simulink model "zsi_mppt_grid_pv"  (R2024b)
settings: Solver=FixedStepDiscrete  StartTime=0.0  StopTime=5  FixedStep=1e-6  RelTol=1e-3
libraries: spsSeriesRLCBranchLib x5, spsDiodeLib x4, spsVoltageMeasurementLib x4, spsPVArrayLib x3, dspstat3 x2, spsCurrentMeasurementLib x1, simulink x1, spsThreePhaseSeriesRLCBranchLib x1, spsThreePhaseVIMeasurementLib x1, spsThreePhaseSourceLib x1, spsUniversalBridgeLib x1, sps_lib x1
settings Model: Creator=Dhananjay Dhumal  LastModifiedBy=Dhananjay Dhumal
settings DebuggingCC: SignalInfNanChecking=error

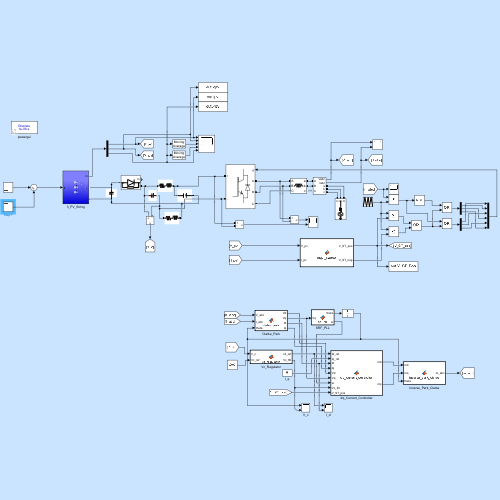
[thumbnail: Simulink's stored preview of the top-level diagram]
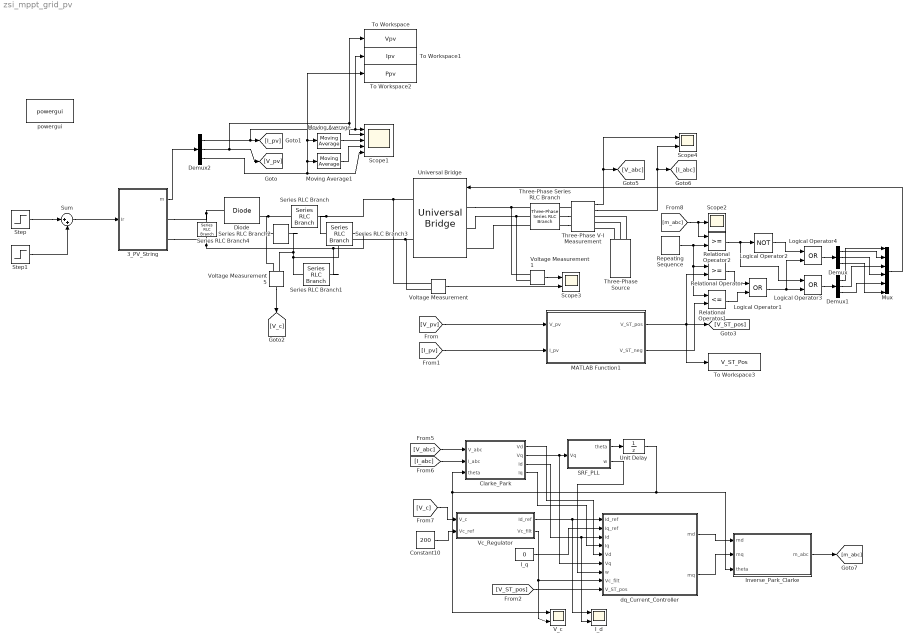
== system zsi_mppt_grid_pv ==
  3_PV_String : Subsystem
  Clarke_Park : MATLAB Function  TreatAsAtomicUnit=on
  Constant10 : Constant  Value=200
  Demux : Demux  Outputs=3
  Demux1 : Demux  Outputs=3
  Demux2 : Demux  Outputs=3
  Diode : spsDiodeLib/Diode  Ron=0.001  Lon=0  Vf=0.8  IC=0  UseSnubber=0  Rs=500  Cs=250e-9  Measurements=on
  I_d : Scope  NumInputPorts=2
  I_q : Constant  Value=0
  Inverse_Park_Clarke : MATLAB Function  TreatAsAtomicUnit=on
  Logical Operator1 : Logic  Operator=OR  AllPortsSameDT=off  OutDataTypeStr=boolean
  Logical Operator2 : Logic  Operator=NOT  AllPortsSameDT=off  OutDataTypeStr=boolean
  Logical Operator3 : Logic  Operator=OR  AllPortsSameDT=off  OutDataTypeStr=boolean
  Logical Operator4 : Logic  Operator=OR  AllPortsSameDT=off  OutDataTypeStr=boolean
  MATLAB Function1 : MATLAB Function  TreatAsAtomicUnit=on
  Moving Average : dspstat3/Moving Average  Method=Sliding window  ForgettingFactorPort=off  SpecifyWindowLength=on  WindowLength=500  OverlapLength=499  AllowArbitraryInputLength=off  ForgettingFactor=0.9  SimulateUsing=Interpreted execution
  Moving Average1 : dspstat3/Moving Average  Method=Sliding window  ForgettingFactorPort=off  SpecifyWindowLength=on  WindowLength=10000  OverlapLength=9999  AllowArbitraryInputLength=off  ForgettingFactor=0.9  SimulateUsing=Interpreted execution
  Mux : Mux  Inputs=6
  Relational Operator : RelationalOperator  OutDataTypeStr=boolean  RndMeth=Simplest  InputSameDT=off
  Relational Operator1 : RelationalOperator  Operator=<=  OutDataTypeStr=boolean  RndMeth=Simplest  InputSameDT=off
  Relational Operator2 : RelationalOperator  OutDataTypeStr=boolean  RndMeth=Simplest  InputSameDT=off
  Repeating Sequence : simulink/Sources/Repeating Sequence  rep_seq_t=[0 0.5e-4 1e-4]  rep_seq_y=[-1 1 -1]
  SRF_PLL : MATLAB Function  TreatAsAtomicUnit=on
  Scope1 : Scope  NumInputPorts=5
  Scope2 : Scope
  Scope3 : Scope  NumInputPorts=2
  Scope4 : Scope  NumInputPorts=2
  Series RLC Branch : spsSeriesRLCBranchLib/Series RLC Branch  LConnTagsString=__new0  RConnTagsString=__new0  BranchType=RL  Resistance=0.2  Inductance=1e-3  SetiL0=off  InitialCurrent=0  Capacitance=1e-6  Setx0=off  InitialVoltage=0  Measurements=None
  Series RLC Branch1 : spsSeriesRLCBranchLib/Series RLC Branch  LConnTagsString=__new0  RConnTagsString=__new0  BranchType=RL  Resistance=0.2  Inductance=1e-3  SetiL0=off  InitialCurrent=0  Capacitance=1e-6  Setx0=off  InitialVoltage=0  Measurements=None
  Series RLC Branch2 : spsSeriesRLCBranchLib/Series RLC Branch  LConnTagsString=__new0  RConnTagsString=__new0  BranchType=C  Resistance=1  Inductance=1e-3  SetiL0=off  InitialCurrent=0  Capacitance=1000e-6  Setx0=on  InitialVoltage=200  Measurements=None
  Series RLC Branch3 : spsSeriesRLCBranchLib/Series RLC Branch  LConnTagsString=__new0  RConnTagsString=__new0  BranchType=C  Resistance=1  Inductance=1000e-3  SetiL0=off  InitialCurrent=0  Capacitance=1000e-6  Setx0=on  InitialVoltage=200  Measurements=None
  Series RLC Branch4 : spsSeriesRLCBranchLib/Series RLC Branch  LConnTagsString=__new0  RConnTagsString=__new0  BranchType=C  Resistance=1  Inductance=1e-3  SetiL0=off  InitialCurrent=0  Capacitance=150e-6  Setx0=on  InitialVoltage=192  Measurements=None
  Step : Step  Time=1.5  Before=[1000, 1000, 1000]  After=[1000, 700, 350]  SampleTime=0
  Step1 : Step  Time=3.5  Before=[0, 0, 0]  After=[-800, -200, 700]  SampleTime=0
  Sum : Sum  Inputs=|++
  Three-Phase Series RLC Branch : spsThreePhaseSeriesRLCBranchLib/Three-Phase Series RLC Branch  LConnTagsString=A|B|C  RConnTagsString=A|B|C  BranchType=L  Resistance=1  Inductance=5e-3  Capacitance=1e-6  Measurements=None
  Three-Phase V-I Measurement : spsThreePhaseVIMeasurementLib/Three-Phase V-I Measurement  VoltageMeasurement=phase-to-ground  SetLabelV=off  LabelV=Vabc  Vpu=off  VpuLL=off  CurrentMeasurement=yes  SetLabelI=off  LabelI=Iabc  Ipu=off  Pbase=100e6  Vbase=500e3  OutputType=Complex  PhasorSimulation=off  PSBequivalent=0
  Three-Phase Source : spsThreePhaseSourceLib/Three-Phase Source  InternalConnection=Yg  VoltagePhases=off  Voltage=100  PhaseAngle=0  Voltage_phases=[25e3 25e3 25e3]/sqrt(3)  PhaseAngles_phases=[0 -120 +120]  Frequency=50  NonIdealSource=on  SpecifyImpedance=off  Resistance=0.001  Inductance=0  ShortCircuitLevel=100e6  BaseVoltage=100  XRratio=7  BusType=swing  Pref=10e3  Qref=0  Prefabc=[10e3, 10e3, 10e3]  Qrefabc=[0, 0, 0]  Qmin=-inf  Qmax=inf
  To Workspace : ToWorkspace  VariableName=Vpv  SaveFormat=Timeseries  SampleTime=-1
  To Workspace1 : ToWorkspace  VariableName=Ipv  SaveFormat=Timeseries  SampleTime=-1
  To Workspace2 : ToWorkspace  VariableName=Ppv  SaveFormat=Timeseries  SampleTime=-1
  To Workspace3 : ToWorkspace  VariableName=V_ST_Pos  SaveFormat=Timeseries  SampleTime=-1
  Unit Delay : UnitDelay  SampleTime=1e-6  HasFrameUpgradeWarning=on
  Universal Bridge : spsUniversalBridgeLib/Universal Bridge  Arms=3  SnubberResistance=1e5  SnubberCapacitance=inf  Device=IGBT / Diodes  Ron=1e-3  Lon=0  ForwardVoltages="[  0  0  ]"  ForwardVoltage=0  GTOparameters=[ 10e-6 , 20e-6 ]  IGBTparameters=[ 1e-6 , 2e-6 ]  Measurements=All voltages and currents  Measurements_2=None  converterType=Rectifier
  V_c : Scope  NumInputPorts=2
  Vc_Regulator : MATLAB Function  TreatAsAtomicUnit=on
  Voltage Measurement : spsVoltageMeasurementLib/Voltage Measurement  PhasorSimulation=off  OutputType=Complex  PSBequivalent=0
  Voltage Measurement1 : spsVoltageMeasurementLib/Voltage Measurement  PhasorSimulation=off  OutputType=Complex  PSBequivalent=0
  Voltage Measurement5 : spsVoltageMeasurementLib/Voltage Measurement  PhasorSimulation=off  OutputType=Complex  PSBequivalent=0
  dq_Current_Controller : MATLAB Function  TreatAsAtomicUnit=on
  powergui : sps_lib/powergui  Priority=1  SimulationMode=Discrete  SampleTime=1e-6  frequency=60  Iterations=50  frequencyindice=0  Pbase=100e6  ErrMax=1e-4  UnitsV=kV  UnitsW=MW  buscounter=0  FunctionMessages=off  echomessages=off  EnableUseOfTLC=off  CurrentSourceSwitches=off  DisableSnubberDevices=off  DisableRonSwitches=off  DisableVfSwitches=off  DisplayEquations=off  AutomaticDiscreteSolvers=off  SolverType=Tustin/Backward Euler (TBE)  Interpol=off  ExternalGateDelay=off  methode=off  Ts=100  x0status=blocks  SPID=on  SwTol=0  HookPort=off  NonlinearTolerance=1e-4  nMaxIteration=100  ContinueOnMaxIteration=off  RestoreLinks=warning  ResistiveCurrentMeasurement=off  Frange=[0:2:500]  Ylog=off  Xlog=on  ShowGrid=off  save=off  variable=ZData  structure=0  ZoomFFT=off  StartTime=0.0  cycles=1  DisplayStyle=1  fundamental=60  FreqAxis=off  MaxFrequency=1000  frequencyindicesteady=1  RmsSteady=1  display=off
  wires:
  Voltage Measurement/1 -> Scope3/2
  Repeating Sequence/1 -> Relational Operator2/2, Relational Operator/1, Relational Operator1/1
  Relational Operator/1 -> Logical Operator1/1
  Relational Operator1/1 -> Logical Operator1/2
  Logical Operator1/1 -> Logical Operator4/2, Logical Operator3/2
  Logical Operator4/1 -> Demux/1
  Logical Operator3/1 -> Demux1/1
  Voltage Measurement1/1 -> Scope3/1
  MATLAB Function1/1(V_ST_pos) -> To Workspace3/1, Relational Operator/2, [V_ST_pos]
  MATLAB Function1/2(V_ST_neg) -> Relational Operator1/2
  Voltage Measurement5/1 -> [V_c]
  Three-Phase V-I Measurement/1 -> Scope4/1, [V_abc]
  Three-Phase V-I Measurement/2 -> Scope4/2, [I_abc]
  [V_abc] -> Clarke_Park/1(V_abc)
  [I_abc] -> Clarke_Park/2(I_abc)
  Clarke_Park/2(Vq) -> dq_Current_Controller/6(Vq), SRF_PLL/1(Vq)
  SRF_PLL/1(theta) -> Unit Delay/1
  Unit Delay/1 -> V_c/1, Clarke_Park/3(theta), Inverse_Park_Clarke/3(theta)
  [V_c] -> Vc_Regulator/1(V_c)
  Constant10/1 -> Vc_Regulator/2(Vc_ref)
  Vc_Regulator/1(Id_ref) -> I_d/1, dq_Current_Controller/1(Id_ref)
  I_q/1 -> dq_Current_Controller/2(Iq_ref)
  Clarke_Park/3(Id) -> I_d/2, dq_Current_Controller/3(Id)
  Clarke_Park/4(Iq) -> dq_Current_Controller/4(Iq)
  Clarke_Park/1(Vd) -> dq_Current_Controller/5(Vd)
  SRF_PLL/2(w) -> dq_Current_Controller/7(w)
  Vc_Regulator/2(Vc_filt) -> V_c/2, dq_Current_Controller/8(Vc_filt)
  dq_Current_Controller/1(md) -> Inverse_Park_Clarke/1(md)
  dq_Current_Controller/2(mq) -> Inverse_Park_Clarke/2(mq)
  Inverse_Park_Clarke/1(m_abc) -> [m_abc]
  [m_abc] -> Scope2/1, Relational Operator2/1
  [V_ST_pos] -> dq_Current_Controller/9(V_ST_pos)
  [V_pv] -> MATLAB Function1/1(V_pv)
  [I_pv] -> MATLAB Function1/2(I_pv)
  Mux/1 -> Universal Bridge/1
  Relational Operator2/1 -> Logical Operator3/1, Logical Operator2/1
  Demux/1 -> Mux/2
  Demux/2 -> Mux/4
  Demux/3 -> Mux/6
  Demux1/1 -> Mux/1
  Demux1/2 -> Mux/3
  Demux1/3 -> Mux/5
  Logical Operator2/1 -> Logical Operator4/1
  Step/1 -> Sum/1
  3_PV_String/1(m) -> Demux2/1
  Demux2/1 -> To Workspace1/1, Scope1/1, [I_pv]
  Demux2/2 -> To Workspace/1, Scope1/2, [V_pv]
  Demux2/3 -> To Workspace2/1, Moving Average/1, Moving Average1/1, Scope1/5
  Moving Average/1 -> Scope1/3
  Moving Average1/1 -> Scope1/4
  Sum/1 -> 3_PV_String/1(Ir)
  Step1/1 -> Sum/2
  connections:
  Series RLC Branch/LConn1 -- Series RLC Branch2/LConn1 -- Voltage Measurement5/LConn1 -- Diode/RConn1
  Series RLC Branch3/RConn1 -- Series RLC Branch1/RConn1 -- 3_PV_String/RConn2 -- Series RLC Branch4/RConn1
  Series RLC Branch2/RConn1 -- Series RLC Branch1/LConn1 -- Voltage Measurement/LConn2 -- Universal Bridge/RConn2 -- Voltage Measurement5/LConn2
  Series RLC Branch/RConn1 -- Series RLC Branch3/LConn1 -- Universal Bridge/RConn1 -- Voltage Measurement/LConn1
  Universal Bridge/LConn1 -- Three-Phase Series RLC Branch/LConn1 -- Voltage Measurement1/LConn1
  Voltage Measurement1/LConn2 -- Three-Phase Series RLC Branch/LConn2 -- Universal Bridge/LConn2
  Three-Phase Series RLC Branch/LConn3 -- Universal Bridge/LConn3
  Three-Phase V-I Measurement/LConn1 -- Three-Phase Series RLC Branch/RConn1
  Three-Phase Series RLC Branch/RConn3 -- Three-Phase V-I Measurement/LConn3
  Three-Phase Series RLC Branch/RConn2 -- Three-Phase V-I Measurement/LConn2
  Three-Phase Source/RConn2 -- Three-Phase V-I Measurement/RConn2
  Three-Phase Source/RConn1 -- Three-Phase V-I Measurement/RConn1
  Three-Phase Source/RConn3 -- Three-Phase V-I Measurement/RConn3
  3_PV_String/RConn1 -- Diode/LConn1 -- Series RLC Branch4/LConn1

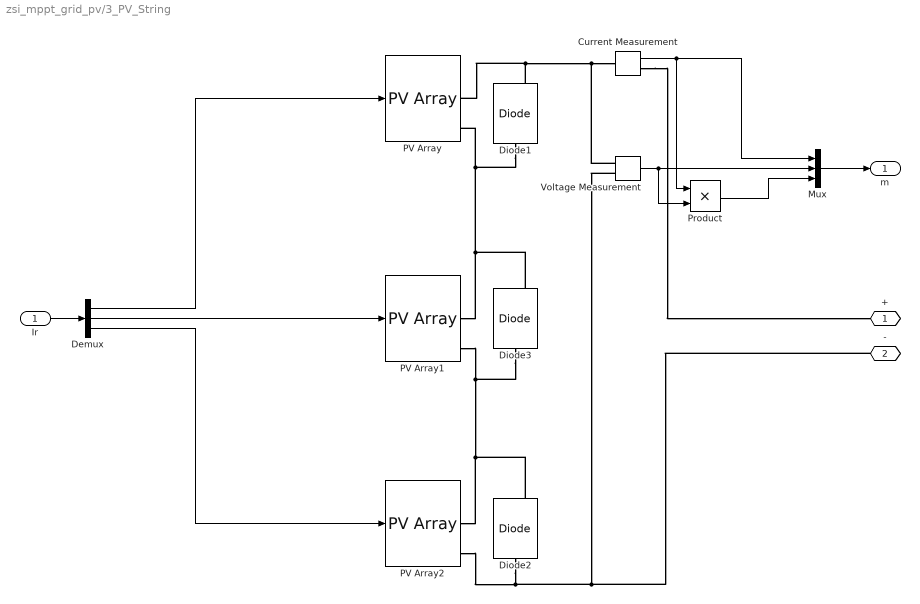
== system zsi_mppt_grid_pv/3_PV_String ==
  Ir : Inport  PortDimensions=3
  Current Measurement : spsCurrentMeasurementLib/Current Measurement  PhasorSimulation=off  OutputType=Complex  PSBequivalent=0
  Demux : Demux  Outputs=3
  Diode1 : spsDiodeLib/Diode  Ron=1e-5  Lon=0  Vf=0  IC=0  UseSnubber=0  Rs=1e5  Cs=inf  Measurements=on
  Diode2 : spsDiodeLib/Diode  Ron=1e-5  Lon=0  Vf=0  IC=0  UseSnubber=0  Rs=1e5  Cs=inf  Measurements=on
  Diode3 : spsDiodeLib/Diode  Ron=1e-5  Lon=0  Vf=0  IC=0  UseSnubber=0  Rs=1e5  Cs=inf  Measurements=on
  Mux : Mux  Inputs=3
  PV Array : spsPVArrayLib/PV Array  Npar=1  Nser=1  PlotType=array @ 1000 W/m2 & specified temperatures  S_vec="[ 1000  500  100 ]"  Temp_C_vec="[ 45 25  ]"  ModuleName=SunPower SPR-305E-WHT-D  PlotWhenSelected=off  Pm=305.226  Ncell=96  Voc=64.2  Isc=5.96  Vm=54.7  Im=5.58  beta_Voc_pc=-0.2727  alpha_Isc_pc=0.061745  beta_Voc=-0.17507  alpha_Isc=0.00368  IL=5.9657  I0=6.3076e-12  nI=0.94489  Rsh=393.2054  Rs=0.37428  RobustModel=on  RobustCellTemperature=25  BAL=on  Tc=1e-6  Tfilter=5e-5
  PV Array1 : spsPVArrayLib/PV Array  Npar=1  Nser=1  PlotType=array @ 1000 W/m2 & specified temperatures  S_vec="[ 1000  500  100 ]"  Temp_C_vec="[ 45 25  ]"  ModuleName=SunPower SPR-305E-WHT-D  PlotWhenSelected=off  Pm=305.226  Ncell=96  Voc=64.2  Isc=5.96  Vm=54.7  Im=5.58  beta_Voc_pc=-0.2727  alpha_Isc_pc=0.061745  beta_Voc=-0.17507  alpha_Isc=0.00368  IL=5.9657  I0=6.3076e-12  nI=0.94489  Rsh=393.2054  Rs=0.37428  RobustModel=on  RobustCellTemperature=25  BAL=on  Tc=1e-6  Tfilter=5e-5
  PV Array2 : spsPVArrayLib/PV Array  Npar=1  Nser=1  PlotType=array @ 1000 W/m2 & specified temperatures  S_vec="[ 1000  500  100 ]"  Temp_C_vec="[ 45 25  ]"  ModuleName=SunPower SPR-305E-WHT-D  PlotWhenSelected=off  Pm=305.226  Ncell=96  Voc=64.2  Isc=5.96  Vm=54.7  Im=5.58  beta_Voc_pc=-0.2727  alpha_Isc_pc=0.061745  beta_Voc=-0.17507  alpha_Isc=0.00368  IL=5.9657  I0=6.3076e-12  nI=0.94489  Rsh=393.2054  Rs=0.37428  RobustModel=on  RobustCellTemperature=25  BAL=on  Tc=1e-6  Tfilter=5e-5
  Product : Product
  Voltage Measurement : spsVoltageMeasurementLib/Voltage Measurement  PhasorSimulation=off  OutputType=Complex  PSBequivalent=0
  + : PMIOPort  Side=Right
  - : PMIOPort  Port=2  Side=Right
  m : Outport  PortDimensions=3
  wires:
  Ir/1 -> Demux/1
  Demux/1 -> PV Array/1
  Demux/2 -> PV Array1/1
  Demux/3 -> PV Array2/1
  Mux/1 -> m/1
  Current Measurement/1 -> Mux/1, Product/1
  Voltage Measurement/1 -> Product/2, Mux/2
  Product/1 -> Mux/3
  connections:
  Diode3/LConn1 -- PV Array1/RConn2 -- PV Array2/RConn1 -- Diode2/RConn1
  Diode3/RConn1 -- PV Array1/RConn1 -- Diode1/LConn1 -- PV Array/RConn2
  PV Array/RConn1 -- Diode1/RConn1 -- Voltage Measurement/LConn1 -- Current Measurement/LConn1
  Diode2/LConn1 -- -/RConn1 -- Voltage Measurement/LConn2 -- PV Array2/RConn2
  Current Measurement/RConn1 -- +/RConn1

== matlab function zsi_mppt_grid_pv/MATLAB Function1 ==
  data: V_pv input; V_ST_pos output; I_pv input; V_ST_neg output
function [V_ST_pos, V_ST_neg] = mppt_sweep(V_pv, I_pv)
    persistent state timer D_0 P_max D_max sweep_delay V_sum I_sum count
    
    if isempty(state)
        state = 0;
        timer = 0;
        D_0 = 0.0;
        P_max = 0;
        D_max = 0;
        sweep_delay = 0;
        V_sum = 0;
        I_sum = 0;
        count = 0;
    end
    
    % State 0: Hold at GMPP for 0.5 seconds (500,000 steps at 1 us)
    if state == 0
        timer = timer + 1;
        if timer > 500000 
            state = 1;
            timer = 0;
            D_0 = 0.0; 
            P_max = 0;
            sweep_delay = 0;
            V_sum = 0;
            I_sum = 0;
            count = 0;
        end
        
    % State 1: 13-step staircase sweep (steps of 0.02 held for 10 ms = 10,000 steps each)
    elseif state == 1
        sweep_delay = sweep_delay + 1;
        
        % First 5 ms (1..5000): let the LC step transient settle completely
        % Last 5 ms (5001..10000): accumulate true average V_pv and I_pv
        if sweep_delay > 5000
            V_sum = V_sum + V_pv;
            I_sum = I_sum + I_pv;
            count = count + 1;
        end
        
        % At the end of the 10 ms step, compute settled average power and advance D_0
        if sweep_delay >= 10000
            V_avg = V_sum / max(count, 1);
            I_avg = I_sum / max(count, 1);
            P_pv = V_avg * I_avg;
            
            if P_pv > P_max
                P_max = P_pv;
                D_max = D_0;
            end
            
            D_0 = D_0 + 0.02; 
            sweep_delay = 0;
            V_sum = 0;
            I_sum = 0;
            count = 0;
        end
        
        if D_0 > 0.25
            state = 0;
            D_0 = D_max; 
        end
    end
    
    % Staggered thresholds for 13 distinct physical steps at 10 kHz / 1 us
    V_ST_pos = 1 - D_0;
    V_ST_neg = -1 + max(D_0 - 0.02, 0);
end

== matlab function zsi_mppt_grid_pv/Clarke_Park ==
  data: V_abc input; Vd output; I_abc input; theta input; Vq output; Id output; Iq output
function [Vd, Vq, Id, Iq] = clarke_park(V_abc, I_abc, theta)
    % Sine-aligned Clarke + Park Transform (abc -> dq)
    sa = sin(theta);
    sb = sin(theta - 2*pi/3);
    sc = sin(theta + 2*pi/3);
    ca = cos(theta);
    cb = cos(theta - 2*pi/3);
    cc = cos(theta + 2*pi/3);
    
    Vd = (2/3) * (V_abc(1)*sa + V_abc(2)*sb + V_abc(3)*sc);
    Vq = (2/3) * (V_abc(1)*ca + V_abc(2)*cb + V_abc(3)*cc);
    
    Id = (2/3) * (I_abc(1)*sa + I_abc(2)*sb + I_abc(3)*sc);
    Iq = (2/3) * (I_abc(1)*ca + I_abc(2)*cb + I_abc(3)*cc);
end

== matlab function zsi_mppt_grid_pv/SRF_PLL ==
  data: Vq input; theta output; w output
function [theta, w] = srf_pll(Vq)
    persistent theta_state int_pll
    Ts = 1e-6; % Updated to 1 us
    w0 = 2 * pi * 50; 
    Kp_pll = 100;
    Ki_pll = 2000;
    
    if isempty(theta_state)
        theta_state = 0;
        int_pll = 0;
    end
    
    int_pll = max(min(int_pll + Ki_pll * Vq * Ts, 30), -30);
    w = max(min(w0 + Kp_pll * Vq + int_pll, 2*pi*55), 2*pi*45);
    theta_state = mod(theta_state + w * Ts, 2*pi);
    
    theta = theta_state;
end

== matlab function zsi_mppt_grid_pv/Vc_Regulator ==
  data: V_c input; Id_ref output; Vc_ref input; Vc_filt output
function [Id_ref, Vc_filt] = vc_regulator(V_c, Vc_ref)
    persistent Vc_state int_vc
    Ts = 1e-6; % Updated to 1 us
    Kp_vc = 0.4;
    Ki_vc = 15.0;
    
    if isempty(Vc_state)
        Vc_state = 200;
        int_vc = 0;
    end
    
    % 2 ms low-pass filter scaled for Ts = 1e-6
    Vc_state = 0.9995 * Vc_state + 0.0005 * V_c;
    Vc_filt = Vc_state;
    
    err_vc = Vc_filt - Vc_ref;
    
    int_vc = int_vc + Ki_vc * err_vc * Ts;
    int_vc = max(min(int_vc, 15), 0);
    
    Id_ref = max(min(Kp_vc * err_vc + int_vc, 15), 0);
end

== matlab function zsi_mppt_grid_pv/dq_Current_Controller ==
  data: Id_ref input; md output; Iq_ref input; Id input; Iq input; Vd input; Vq input; w input; Vc_filt input; V_ST_pos input; mq output
function [md, mq] = dq_current_controller(Id_ref, Iq_ref, Id, Iq, Vd, Vq, w, Vc_filt, V_ST_pos)
    persistent int_id int_iq
    Ts = 1e-6;
    L_grid = 5e-3;
    Kp_i = 2.0;   % Damped proportional gain for pure L filter (R = 0)
    Ki_i = 50.0;  % Smooth integral gain
    
    if isempty(int_id)
        int_id = 0;
        int_iq = 0;
    end
    
    err_id = Id_ref - Id;
    err_iq = Iq_ref - Iq;
    
    int_id = max(min(int_id + Ki_i * err_id * Ts, 10), -10);
    int_iq = max(min(int_iq + Ki_i * err_iq * Ts, 10), -10);
    
    % Bound the PI correction to +/- 15V around the exact grid voltage Vd, Vq
    u_d = max(min(Kp_i * err_id + int_id, 15), -15);
    u_q = max(min(Kp_i * err_iq + int_iq, 15), -15);
    
    Vd_conv = Vd - w * L_grid * Iq + u_d;
    Vq_conv = Vq + w * L_grid * Id + u_q;
    
    % Normalize by active Z-source DC bus voltage
    V_base = max(Vc_filt, 180) / (2 * max(V_ST_pos, 0.7));
    md = Vd_conv / V_base;
    mq = Vq_conv / V_base;
    
    % Enforce Simple Boost Control limit: M <= 0.95 * (1 - D_0)
    M_mag = sqrt(md^2 + mq^2);
    M_max = 0.95 * V_ST_pos;
    if M_mag > M_max && M_mag > 0
        md = md * (M_max / M_mag);
        mq = mq * (M_max / M_mag);
    end
end

== matlab function zsi_mppt_grid_pv/Inverse_Park_Clarke ==
  data: md input; m_abc output; mq input; theta input
function m_abc = inverse_park_clarke(md, mq, theta)
    % Sine-aligned Inverse Park Transform
    sa = sin(theta);
    sb = sin(theta - 2*pi/3);
    sc = sin(theta + 2*pi/3);
    ca = cos(theta);
    cb = cos(theta - 2*pi/3);
    cc = cos(theta + 2*pi/3);
    
    ma = md * sa + mq * ca;
    mb = md * sb + mq * cb;
    mc = md * sc + mq * cc;
    
    m_abc = [ma; mb; mc];
end
